simulink model "LineFollowerPID"  (R2024b)
settings: Solver=FixedStepDiscrete  StartTime=0.0  StopTime=30  FixedStep=0.001  RelTol=1e-3
model workspace (MAT data in the model file):
  Kp = 5
  baseSpeed = 90
settings Model: Creator=Devansh  LastModifiedBy=Devansh

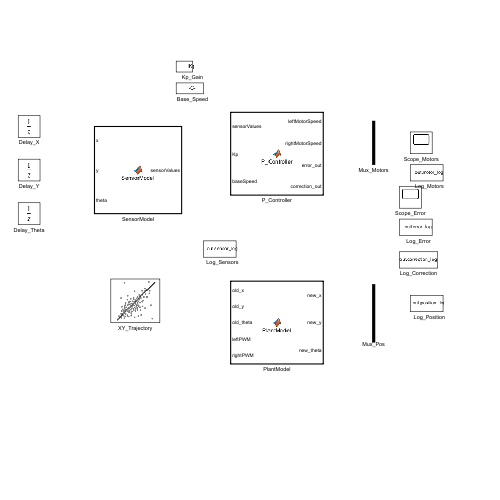
[thumbnail: Simulink's stored preview of the top-level diagram]
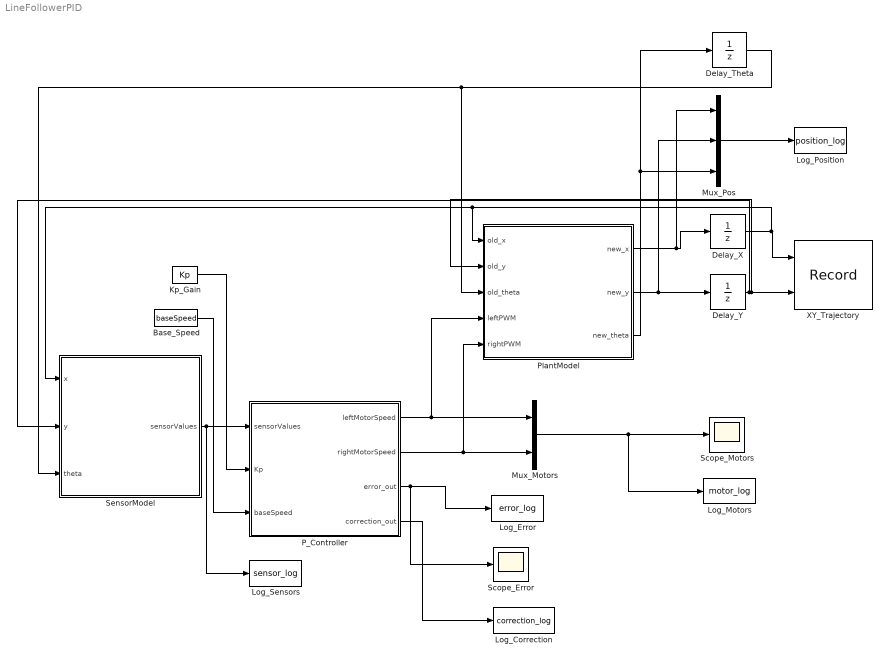
== system LineFollowerPID ==
  Base_Speed : Constant  Value=baseSpeed
  Delay_Theta : UnitDelay  SampleTime=-1  HasFrameUpgradeWarning=on
  Delay_X : UnitDelay  SampleTime=-1  HasFrameUpgradeWarning=on
  Delay_Y : UnitDelay  SampleTime=-1  HasFrameUpgradeWarning=on
  Kp_Gain : Constant  Value=Kp
  Log_Correction : ToWorkspace  VariableName=correction_log  SampleTime=-1
  Log_Error : ToWorkspace  VariableName=error_log  SampleTime=-1
  Log_Motors : ToWorkspace  VariableName=motor_log  SampleTime=-1
  Log_Position : ToWorkspace  VariableName=position_log  SampleTime=-1
  Log_Sensors : ToWorkspace  VariableName=sensor_log  SampleTime=-1
  Mux_Motors : Mux  Inputs=2
  Mux_Pos : Mux  Inputs=3
  P_Controller : MATLAB Function  TreatAsAtomicUnit=on
  PlantModel : MATLAB Function  TreatAsAtomicUnit=on
  Scope_Error : Scope
  Scope_Motors : Scope
  SensorModel : MATLAB Function  TreatAsAtomicUnit=on
  XY_Trajectory : Record  FileSettingsInternal="{\"entries\":[{\"content\":{\"excelSettings\":{\"content\":{},\"type\":\"Streamout.ExcelSettings\"}},\"type\":\"Streamout.FileSettingStorage\",\"uuid\":\"\"}],\"packageUris\":[\"http:\\/\\/schema.mathworks.com\\/mf0\\/streamout_blocks\\/R2020a\"],\"version\":\"1.0\"}"  Layout=[1 1]  SignalsInternal="{\"entries\":[{\"content\":{\"signals\":[{\"content\":{\"blockPath\":[],\"dimensions\":[1],\"domain\":\"\",\"lineColor\":\"#a2142f\",\"plots\":[ 1 ],\"port\":1,\"signalID\":1,\"signalName\":\"XY Graph:1\"},\"type\":\"RecordBlkView.Signal\",\"uuid\":\"\"},{\"content\":{\"blockPath\":[],\"dimensions\":[1],\"domain\":\"\",\"lineColor\":\"#139fff\",\"plots\":[ 1 ],\"port\":2,\"signalID\":2,\"signalName\":\"XY Graph:2\"},\"type\":\"RecordBlkView.Signal\",\"uuid\":\"\"}]},\"type\":\"RecordBlkView.InputSignals\",\"uuid\":\"\"}],\"packageUris\":[\"http:\\/\\/schema.mathworks.com\\/mf0\\/streamout_blocks\\/R2020a\"],\"version\":\"1.0\"}"  VisualizationBindings="{\"xyplotplugin\":{\"info\":[{\"series\":[{\"bindingParametersList\":[{\"parameter\":\"X-Axis\",\"signalID\":1,\"signalName\":\"XY Graph:1\"},{\"parameter\":\"Y-Axis\",\"signalID\":2,\"signalName\":\"XY Graph:2\"}],\"seriesID\":0}],\"subplotID\":1}]}}"  CompatibilityTag=XY
  wires:
  Base_Speed/1 -> P_Controller/3(baseSpeed)
  Kp_Gain/1 -> P_Controller/2(Kp)
  SensorModel/1(sensorValues) -> P_Controller/1(sensorValues), Log_Sensors/1
  PlantModel/2(new_y) -> Delay_Y/1, Mux_Pos/2
  P_Controller/1(leftMotorSpeed) -> PlantModel/4(leftPWM), Mux_Motors/1
  P_Controller/4(correction_out) -> Log_Correction/1
  P_Controller/3(error_out) -> Scope_Error/1, Log_Error/1
  P_Controller/2(rightMotorSpeed) -> Mux_Motors/2, PlantModel/5(rightPWM)
  PlantModel/1(new_x) -> Mux_Pos/1, Delay_X/1
  PlantModel/3(new_theta) -> Delay_Theta/1, Mux_Pos/3
  Mux_Pos/1 -> Log_Position/1
  Mux_Motors/1 -> Scope_Motors/1, Log_Motors/1
  Delay_Theta/1 -> SensorModel/3(theta), PlantModel/3(old_theta)
  Delay_X/1 -> SensorModel/1(x), PlantModel/1(old_x), XY_Trajectory/1
  Delay_Y/1 -> PlantModel/2(old_y), XY_Trajectory/2, SensorModel/2(y)

== matlab function LineFollowerPID/P_Controller ==
  data: sensorValues input; leftMotorSpeed output; Kp input; baseSpeed input; rightMotorSpeed output; error_out output; correction_out output
function [leftMotorSpeed, rightMotorSpeed, error_out, correction_out] = P_Controller(sensorValues, Kp, baseSpeed)
%#codegen
% =======================================================
%  P-only controller — same sensor processing as Arduino
%  correction = Kp * error   (no I, no D)
% =======================================================

    persistent prevError
    if isempty(prevError)
        prevError = 0;
    end

    % ===== SENSOR PROCESSING (from Arduino code) =====
    weights = [-3, -2, -1, 0, 0, 1, 2, 3];
    position      = 0;
    activeSensors = 0;

    for i = 1:8
        if sensorValues(i) < 900
            binary = 1;
        else
            binary = 0;
        end
        if binary > 0
            activeSensors = activeSensors + 1;
        end
        position = position + binary * weights(i);
    end

    % Lost line protection (uses previous error direction)
    if activeSensors == 0
        if prevError > 0
            position = 12;
        else
            position = -12;
        end
    end

    ir_error  = position / 2.0;
    error_val = ir_error;

    % ===== P-ONLY CONTROL =====
    correction = Kp * error_val;

    prevError = error_val;

    % ===== MOTOR SPEEDS =====
    leftMotorSpeed  = floor(baseSpeed - correction);
    rightMotorSpeed = floor(baseSpeed + correction);
    leftMotorSpeed  = max(-255, min(255, leftMotorSpeed));
    rightMotorSpeed = max(-255, min(255, rightMotorSpeed));

    error_out      = error_val;
    correction_out = correction;
end

== matlab function LineFollowerPID/SensorModel ==
  data: x input; sensorValues output; y input; theta input
function sensorValues = SensorModel(x, y, theta)
%#codegen
    A      = 0.05;
    lambda = 2.0;
    sensorSpacing  = 0.009;
    lineHalfWidth  = 0.010;
    forwardOffset  = 0.06;
    offsets = [-3.5, -2.5, -1.5, -0.5, 0.5, 1.5, 2.5, 3.5] * sensorSpacing;
    sensorValues = zeros(8, 1);
    for i = 1:8
        sx = x + forwardOffset * cos(theta) - offsets(i) * sin(theta);
        sy = y + forwardOffset * sin(theta) + offsets(i) * cos(theta);
        y_track = A * sin(2 * pi * sx / lambda);
        dist = abs(sy - y_track);
        if dist < lineHalfWidth
            sensorValues(i) = 100 + (dist / lineHalfWidth) * 600;
        else
            sensorValues(i) = 1000;
        end
    end
end

== matlab function LineFollowerPID/PlantModel ==
  data: old_x input; new_x output; old_y input; old_theta input; leftPWM input; rightPWM input; new_y output; new_theta output
function [new_x, new_y, new_theta] = PlantModel(old_x, old_y, old_theta, leftPWM, rightPWM)
%#codegen
    dt        = 0.001;
    maxSpeed  = 0.30;
    wheelBase = 0.15;
    v_left  = (leftPWM  / 255.0) * maxSpeed;
    v_right = (rightPWM / 255.0) * maxSpeed;
    v     = (v_left + v_right) / 2.0;
    omega = (v_right - v_left) / wheelBase;
    new_x     = old_x     + v * cos(old_theta) * dt;
    new_y     = old_y     + v * sin(old_theta) * dt;
    new_theta = old_theta + omega * dt;
end
